simulink model "NotebookEdition"  (R2026b)
settings: Solver=FixedStepAuto
libraries: vexv5lib x19, vexcommonlib x1
settings Model: Creator=temporary  LastModifiedBy=temporary
settings OptimizationCC: DefaultParameterBehavior=Inlined  DifferentSizesBufferReuse=on  EfficientTunableParamExpr=on  EnhancedBackFolding=on  MaxStackSize=64  OptimizationCustomize=off  OptimizeBlockOrder=speed  PassReuseOutputArgsAs=Individual arguments  RemoveInternalMemoryZeroInit=on  RemoveRootLevelIOMemoryZeroInit=on
settings DebuggingCC: ParameterTunabilityLossMsg=error
settings HardwareCC: ProdHWDeviceType=ARM Compatible->ARM Cortex  ProdLargestAtomicFloat=Double  ProdLargestAtomicInteger=Long
settings SFSimCC: MATLABDynamicMemAlloc=off
settings RTWCC: Description=Embedded Coder  HardwareBoard=VEX V5 Robot Brain  SystemTargetFile=ert.tlc  TLCOptions="-aInlineSetEventsForThisBaseRateFcn=TLC_FALSE -aSuppressMultiTaskScheduler=TLC_FALSE  -aRateBasedStepFcn=0"  TemplateMakefile=ert_default_tmf  Toolchain=GNU Tools for ARM Embedded Processors
settings CodeAppCC: ForceParamTrailComments=on  IgnoreCustomStorageClasses=off  InsertBlockDesc=on  OperatorAnnotations=on  SFDataObjDesc=on  SimulinkDataObjDesc=on
settings ERTTargetCC: CombineSignalStateStructs=on  ExtModeIntrfLevel=Level2 - Open  ExtModeMexFile=ext_xcp  ExtModeStaticAlloc=on

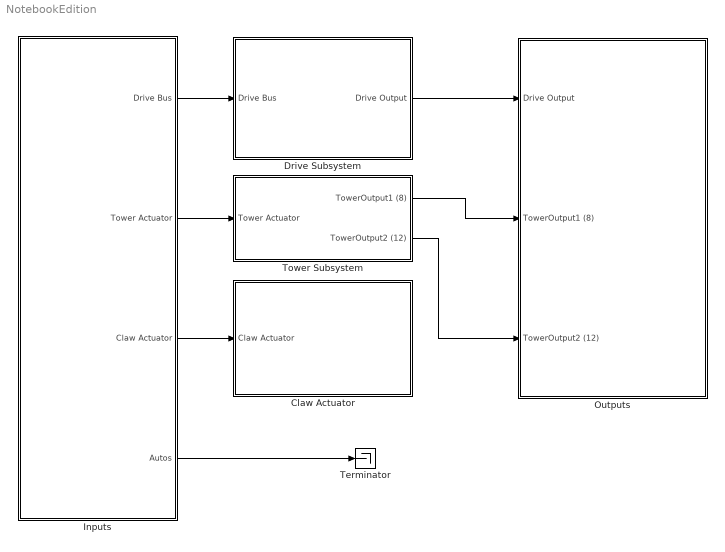
== system NotebookEdition ==
  Claw Actuator : Subsystem
  Drive Subsystem : Subsystem
  Inputs : Subsystem
  Outputs : Subsystem
  Terminator : Terminator
  Tower Subsystem : Subsystem
  wires:
  Inputs/1(Drive Bus) -> Drive Subsystem/1(Drive Bus)
  Inputs/2(Tower Actuator) -> Tower Subsystem/1(Tower Actuator)
  Inputs/3(Claw Actuator) -> Claw Actuator/1(Claw Actuator)
  Inputs/4(Autos) -> Terminator/1
  Drive Subsystem/1(Drive Output) -> Outputs/1(Drive Output)
  Tower Subsystem/1(TowerOutput1 (8)) -> Outputs/2(TowerOutput1 (8))
  Tower Subsystem/2(TowerOutput2 (12)) -> Outputs/3(TowerOutput2 (12))

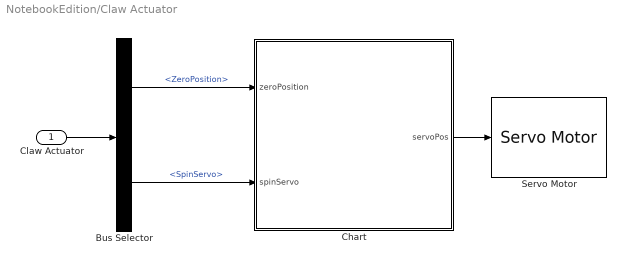
== system NotebookEdition/Claw Actuator ==
  Claw Actuator : Inport
  Bus Selector : BusSelector  OutputSignals=ZeroPosition,SpinServo
  Chart : Stateflow chart  TreatAsAtomicUnit=on
  Servo Motor : vexv5lib/Actuators/Servo Motor  smartPort3wire=15  port=F
  wires:
  Claw Actuator/1 -> Bus Selector/1
  Bus Selector/2 -> Chart/2(spinServo)  "<SpinServo>"
  Bus Selector/1 -> Chart/1(zeroPosition)  "<ZeroPosition>"
  Chart/1(servoPos) -> Servo Motor/1

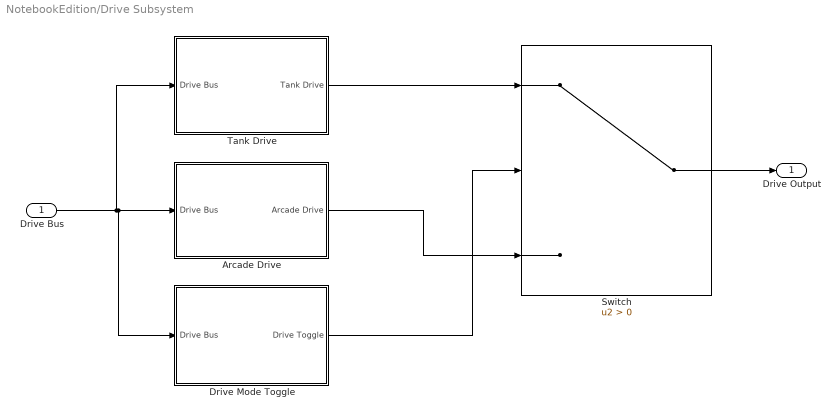
== system NotebookEdition/Drive Subsystem ==
  Drive Bus : Inport
  Arcade Drive : Subsystem
  Drive Mode Toggle : Subsystem
  Switch : Switch  Criteria=u2 > Threshold  SaturateOnIntegerOverflow=off  InputSameDT=off
  Tank Drive : Subsystem
  Drive Output : Outport
  wires:
  Drive Bus/1 -> Drive Mode Toggle/1(Drive Bus), Arcade Drive/1(Drive Bus), Tank Drive/1(Drive Bus)
  Tank Drive/1(Tank Drive) -> Switch/1
  Arcade Drive/1(Arcade Drive) -> Switch/3
  Drive Mode Toggle/1(Drive Toggle) -> Switch/2
  Switch/1 -> Drive Output/1

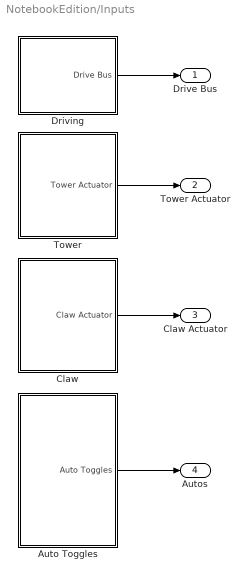
== system NotebookEdition/Inputs ==
  Auto Toggles : Subsystem
  Claw : Subsystem
  Driving : Subsystem
  Tower : Subsystem
  Drive Bus : Outport
  Tower Actuator : Outport  Port=2
  Claw Actuator : Outport  Port=3
  Autos : Outport  Port=4
  wires:
  Driving/1(Drive Bus) -> Drive Bus/1
  Tower/1(Tower Actuator) -> Tower Actuator/1
  Claw/1(Claw Actuator) -> Claw Actuator/1
  Auto Toggles/1(Auto Toggles) -> Autos/1

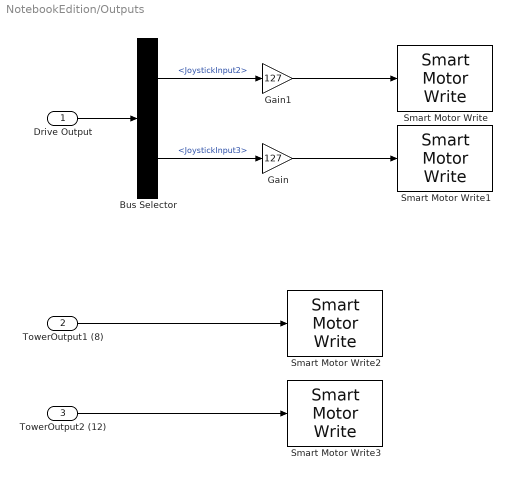
== system NotebookEdition/Outputs ==
  Drive Output : Inport
  TowerOutput1 (8) : Inport  Port=2
  TowerOutput2 (12) : Inport  Port=3
  Bus Selector : BusSelector  OutputSignals=JoystickInput2,JoystickInput3
  Gain : Gain  Gain=127
  Gain1 : Gain  Gain=127
  Smart Motor Write : vexv5lib/Actuators/Smart Motor Write  motorPort=2  scaleFactor=6:1  MotorBrakeMode=Coast  OperationMode=Velocity Control
  Smart Motor Write1 : vexv5lib/Actuators/Smart Motor Write  motorPort=4  scaleFactor=6:1  MotorBrakeMode=Coast  OperationMode=Velocity Control
  Smart Motor Write2 : vexv5lib/Actuators/Smart Motor Write  motorPort=8  scaleFactor=6:1  MotorBrakeMode=Coast  OperationMode=Velocity Control
  Smart Motor Write3 : vexv5lib/Actuators/Smart Motor Write  motorPort=12  scaleFactor=6:1  MotorBrakeMode=Coast  OperationMode=Velocity Control
  wires:
  Drive Output/1 -> Bus Selector/1
  TowerOutput1 (8)/1 -> Smart Motor Write2/1
  TowerOutput2 (12)/1 -> Smart Motor Write3/1
  Bus Selector/2 -> Gain/1  "<JoystickInput3>"
  Gain1/1 -> Smart Motor Write/1
  Bus Selector/1 -> Gain1/1  "<JoystickInput2>"
  Gain/1 -> Smart Motor Write1/1

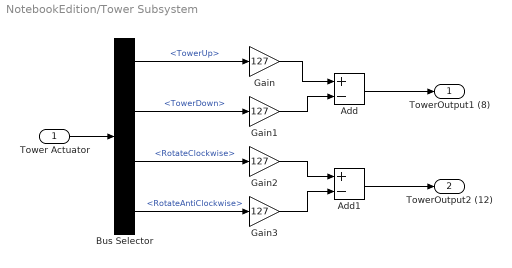
== system NotebookEdition/Tower Subsystem ==
  Tower Actuator : Inport
  Add : Sum  Inputs=+-
  Add1 : Sum  Inputs=+-
  Bus Selector : BusSelector  OutputSignals=TowerUp,TowerDown,RotateClockwise,RotateAntiClockwise
  Gain{,1..3} (4 alike) : Gain  Gain=127
  TowerOutput1 (8) : Outport
  TowerOutput2 (12) : Outport  Port=2
  wires:
  Tower Actuator/1 -> Bus Selector/1
  Bus Selector/4 -> Gain3/1  "<RotateAntiClockwise>"
  Bus Selector/3 -> Gain2/1  "<RotateClockwise>"
  Bus Selector/2 -> Gain1/1  "<TowerDown>"
  Bus Selector/1 -> Gain/1  "<TowerUp>"
  Gain/1 -> Add/1
  Gain1/1 -> Add/2
  Add/1 -> TowerOutput1 (8)/1
  Add1/1 -> TowerOutput2 (12)/1
  Gain2/1 -> Add1/1
  Gain3/1 -> Add1/2

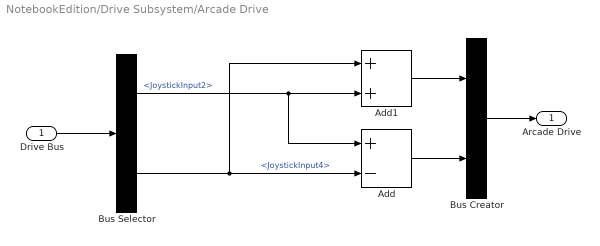
== system NotebookEdition/Drive Subsystem/Arcade Drive ==
  Drive Bus : Inport
  Add : Sum  Inputs=+-
  Add1 : Sum
  Bus Creator : BusCreator  Inputs=2
  Bus Selector : BusSelector  OutputSignals=JoystickInput2,JoystickInput4
  Arcade Drive : Outport
  wires:
  Drive Bus/1 -> Bus Selector/1
  Bus Selector/2 -> Add1/1, Add/2  "<JoystickInput4>"
  Bus Selector/1 -> Add/1, Add1/2  "<JoystickInput2>"
  Add/1 -> Bus Creator/2
  Add1/1 -> Bus Creator/1
  Bus Creator/1 -> Arcade Drive/1

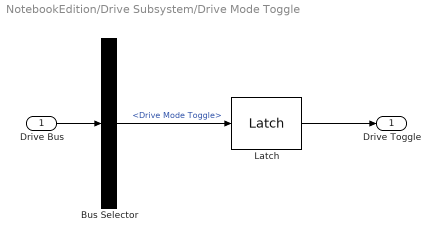
== system NotebookEdition/Drive Subsystem/Drive Mode Toggle ==
  Drive Bus : Inport
  Bus Selector : BusSelector  OutputSignals=Drive Mode Toggle
  Latch : vexcommonlib/Latch  output0=off  BlockPlatform=vexv5
      settings: LibrarySourceBlock=vexv5lib/Utilities/Latch
  Drive Toggle : Outport
  wires:
  Drive Bus/1 -> Bus Selector/1
  Bus Selector/1 -> Latch/1  "<Drive Mode Toggle>"
  Latch/1 -> Drive Toggle/1

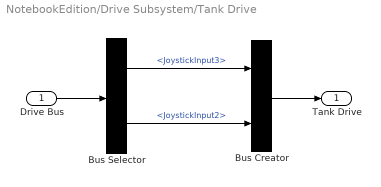
== system NotebookEdition/Drive Subsystem/Tank Drive ==
  Drive Bus : Inport
  Bus Creator : BusCreator  Inputs=2
  Bus Selector : BusSelector  OutputSignals=JoystickInput3,JoystickInput2
  Tank Drive : Outport
  wires:
  Drive Bus/1 -> Bus Selector/1
  Bus Selector/1 -> Bus Creator/1  "<JoystickInput3>"
  Bus Selector/2 -> Bus Creator/2  "<JoystickInput2>"
  Bus Creator/1 -> Tank Drive/1

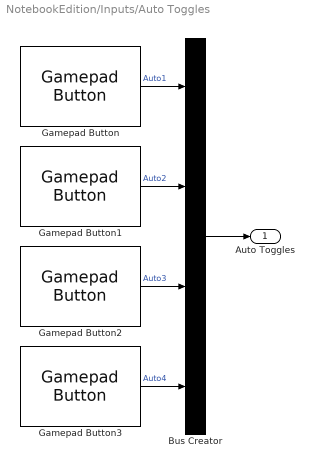
== system NotebookEdition/Inputs/Auto Toggles ==
  Bus Creator : BusCreator  Inputs=4
  Gamepad Button : vexv5lib/Gamepad/Gamepad Button  joystickType=Primary  chan=UP  SampleTime=0.02
  Gamepad Button1 : vexv5lib/Gamepad/Gamepad Button  joystickType=Primary  chan=DOWN  SampleTime=0.02
  Gamepad Button2 : vexv5lib/Gamepad/Gamepad Button  joystickType=Primary  chan=LEFT  SampleTime=0.02
  Gamepad Button3 : vexv5lib/Gamepad/Gamepad Button  joystickType=Primary  chan=RIGHT  SampleTime=0.02
  Auto Toggles : Outport
  wires:
  Gamepad Button/1 -> Bus Creator/1  "Auto1"
  Gamepad Button1/1 -> Bus Creator/2  "Auto2"
  Gamepad Button2/1 -> Bus Creator/3  "Auto3"
  Gamepad Button3/1 -> Bus Creator/4  "Auto4"
  Bus Creator/1 -> Auto Toggles/1

== system NotebookEdition/Inputs/Claw ==
  Bus Creator : BusCreator  Inputs=2
  Gamepad Button : vexv5lib/Gamepad/Gamepad Button  joystickType=Primary  chan=B  SampleTime=0.02
  Gamepad Button2 : vexv5lib/Gamepad/Gamepad Button  joystickType=Primary  chan=X  SampleTime=0.02
  Claw Actuator : Outport
  wires:
  Gamepad Button/1 -> Bus Creator/2  "SpinServo"
  Gamepad Button2/1 -> Bus Creator/1  "ZeroPosition"
  Bus Creator/1 -> Claw Actuator/1

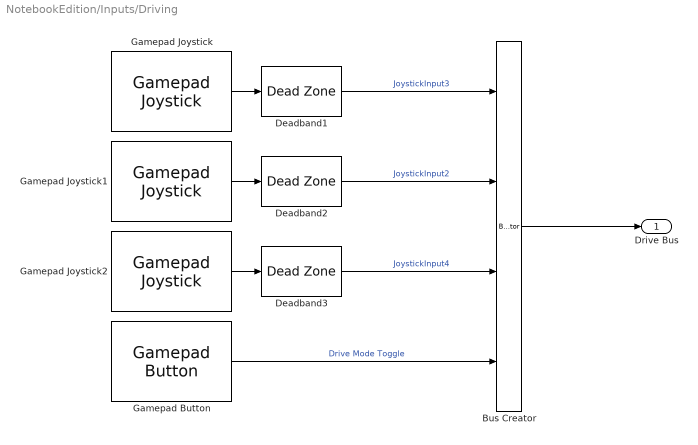
== system NotebookEdition/Inputs/Driving ==
  Bus Creator : BusCreator  Inputs=4
  Deadband1 : DeadZone  LowerValue=-10  UpperValue=10
  Deadband2 : DeadZone  LowerValue=-10  UpperValue=10
  Deadband3 : DeadZone  LowerValue=-10  UpperValue=10
  Gamepad Button : vexv5lib/Gamepad/Gamepad Button  joystickType=Primary  chan=A  SampleTime=0.02
  Gamepad Joystick : vexv5lib/Gamepad/Gamepad Joystick  joystickType=Primary  chan=3  SampleTime=0.02
  Gamepad Joystick1 : vexv5lib/Gamepad/Gamepad Joystick  joystickType=Primary  chan=2  SampleTime=0.02
  Gamepad Joystick2 : vexv5lib/Gamepad/Gamepad Joystick  joystickType=Primary  chan=4  SampleTime=0.02
  Drive Bus : Outport
  wires:
  Gamepad Joystick1/1 -> Deadband2/1
  Gamepad Joystick/1 -> Deadband1/1
  Deadband2/1 -> Bus Creator/2  "JoystickInput2"
  Deadband1/1 -> Bus Creator/1  "JoystickInput3"
  Bus Creator/1 -> Drive Bus/1
  Gamepad Joystick2/1 -> Deadband3/1
  Deadband3/1 -> Bus Creator/3  "JoystickInput4"
  Gamepad Button/1 -> Bus Creator/4  "Drive Mode Toggle"

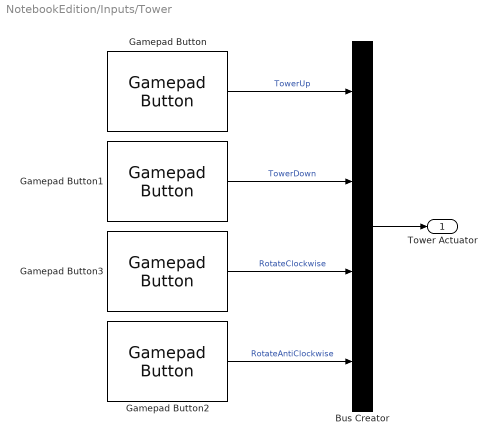
== system NotebookEdition/Inputs/Tower ==
  Bus Creator : BusCreator  Inputs=4
  Gamepad Button : vexv5lib/Gamepad/Gamepad Button  joystickType=Primary  chan=R1  SampleTime=0.02
  Gamepad Button1 : vexv5lib/Gamepad/Gamepad Button  joystickType=Primary  chan=R2  SampleTime=0.02
  Gamepad Button2 : vexv5lib/Gamepad/Gamepad Button  joystickType=Primary  chan=L2  SampleTime=0.02
  Gamepad Button3 : vexv5lib/Gamepad/Gamepad Button  joystickType=Primary  chan=L1  SampleTime=0.02
  Tower Actuator : Outport
  wires:
  Gamepad Button/1 -> Bus Creator/1  "TowerUp"
  Gamepad Button1/1 -> Bus Creator/2  "TowerDown"
  Gamepad Button3/1 -> Bus Creator/3  "RotateClockwise"
  Gamepad Button2/1 -> Bus Creator/4  "RotateAntiClockwise"
  Bus Creator/1 -> Tower Actuator/1

== stateflow chart NotebookEdition/Claw Actuator/Chart ==
  state Mode_Switcher
    entry:
    servoPos = 0;
  state Servo_Spin
    entry:
    servoPos = 90;
  (default) -> Mode_Switcher
  Servo_Spin -> Mode_Switcher : [zeroPosition == 1]
  Mode_Switcher -> Servo_Spin : [spinServo == 1]
  data: zeroPosition input; spinServo input; servoPos output
